simulink model "Unreal3DAnimation"  (R2026a)
settings: Solver=FixedStepAuto  StopTime=inf  FixedStep=0.02
undefined symbols (not defined in the file or in its folder): scenario, Sim3dSensor
libraries: sim3dlib x4, sim3dcameralib x2, dspvision x2, robotsim3dlib x1, visionsinks x1
settings Model: Creator=smaddina  LastModifiedBy=smaddina

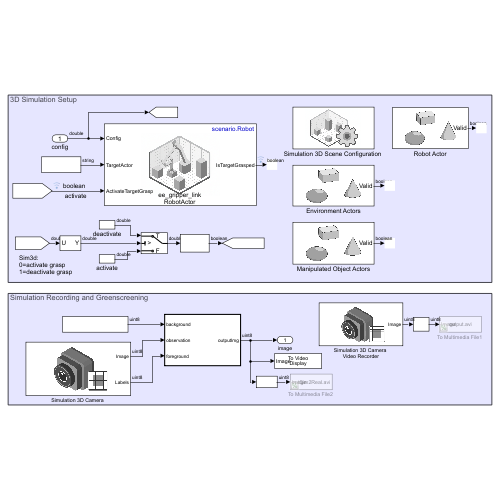
[thumbnail: Simulink's stored preview of the top-level diagram]
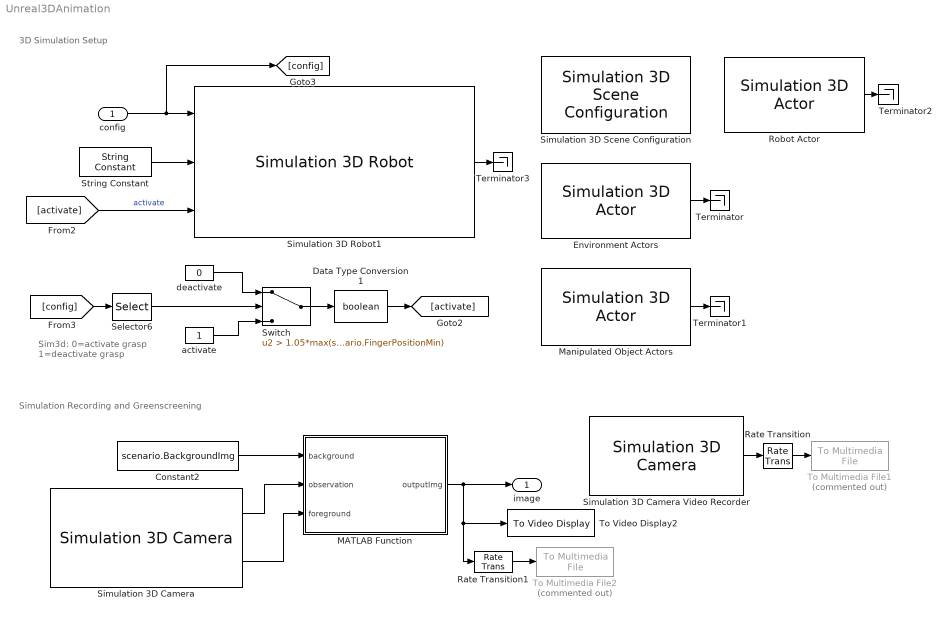
== system Unreal3DAnimation ==
  note: Simulation Recording and Greenscreening
  note: 3D Simulation Setup
  note: Sim3d:
      | 0=activate grasp
      | 1=deactivate grasp
  config : Inport  PortDimensions=scenario.NumConfig
  Constant2 : Constant  Value=scenario.BackgroundImg
  Data Type Conversion1 : DataTypeConversion  OutDataTypeStr=boolean  SaturateOnIntegerOverflow=off  RndMeth=Floor
  Environment Actors : sim3dlib/Simulation 3D Actor  Priority=1  ActorName=Sim3dActor1  ParentName=Scene Origin  Operation=Create at setup  InitScriptText=|  SampleTime=-1  Translation=[0 0 0]  Rotation=[0 0 0]  Scale=single([1 1 1])  aMode=5  ActorTag=Sim3dActor1  ActorType=Sim3dActor  ID=1
      | scenario = evalin("base", "scenario");
      | scenario.setupSceneActor(Actor, World)
  MATLAB Function : MATLAB Function  TreatAsAtomicUnit=on
  Manipulated Object Actors : sim3dlib/Simulation 3D Actor  Priority=1  ActorName=Sim3dActor2  ParentName=Scene Origin  Operation=Create at setup  InitScriptText=|  SampleTime=-1  Translation=[0 0 0]  Rotation=[0 0 0]  Scale=[1 1 1]  aMode=5  ActorTag=Sim3dActor2  ActorType=Sim3dActor  ID=2
      | scenario = evalin("base", "scenario");
      | scenario.setupObjectActor(Actor, World)
  Rate Transition : RateTransition  InitialCondition=zeros(scenario.ImageSize(1),scenario.ImageSize(2),3,'uint8')  OutPortSampleTime=0.2
  Rate Transition1 : RateTransition  InitialCondition=zeros(scenario.ImageSize(1),scenario.ImageSize(2),3,'uint8')  OutPortSampleTime=0.2
  Robot Actor : sim3dlib/Simulation 3D Actor  Priority=1  ActorName=Sim3dActor3  ParentName=Scene Origin  Operation=Create at setup  InitScriptText=|  SampleTime=-1  Translation=[0 0 0]  Rotation=[0 0 0]  Scale=[1 1 1]  aMode=5  ActorTag=Sim3dActor3  ActorType=Sim3dActor  ID=3
      | scenario = evalin("base", "scenario");
      | scenario.setupRobotActor(Actor, World)
  Selector6 : Selector  InputPortWidth=scenario.NumConfig  IndexOptions=Index vector (dialog)  Indices=scenario.FingerLinkIds(1)  OutputSizes=1
  "Simulation 3D Camera " : sim3dcameralib/Simulation 3D Camera  Priority=1  sensorTag=Sim3dSensor�  sensorId=1  sensorName=Sim3dSensor�  vehTagList={'RobotActor';'Scene Origin';'Sim3dActor1';'Sim3dActor2';'base_link'}  vehTag=RobotActor  CoordinateSystem=ISO8855  mountLoc=Origin  offsetFlag=on  tmountOffset=scenario.CameraTransl  extTmount=off  rmountOffset=scenario.CameraRot*180/pi  extRmount=off  FocalLength=scenario.FocalLength  OpticalCenter=scenario.OpticalCenter  ImageSize=scenario.ImageSize  RadialDistortion=[0, 0]  TangentialDistortion=[0, 0]  SensorSkew=0  VisualizeFieldOfView=off  FieldOfViewRange=61  DepthOutportEnabled=off  SemanticOutportEnabled=on  TransformOutportEnabled=off  SampleTime=-1  mountPoint=[0 -0.16 0.336]  mountOrientation=[2.40772307728316e-05 41.8103522312959 26.5650895133509]  aMode=6  ID=1
      settings: LibrarySourceBlock=robotsim3dlib/Simulation 3D Camera
  Simulation 3D Camera Video Recorder : sim3dcameralib/Simulation 3D Camera  Priority=1  sensorTag=Sim3dSensor�  sensorId=2  sensorName=Sim3dSensor�  vehTagList={'Custom ...';'RobotActor';'Scene Origin';'Sim3dActor1';'Sim3dActor2';'Sim3dActor3'}  vehTag=RobotActor  CoordinateSystem=ISO8855  mountLoc=Origin  offsetFlag=on  tmountOffset=scenario.CameraTransl*1.5+[-0.1,0,0]  extTmount=off  rmountOffset=scenario.CameraRot*180/pi  extRmount=off  FocalLength=scenario.FocalLength  OpticalCenter=scenario.OpticalCenter  ImageSize=scenario.ImageSize  RadialDistortion=[0, 0]  TangentialDistortion=[0, 0]  SensorSkew=0  VisualizeFieldOfView=off  FieldOfViewRange=61  DepthOutportEnabled=off  SemanticOutportEnabled=off  TransformOutportEnabled=off  SampleTime=-1  mountPoint=[-0.1 -0.24 0.504]  mountOrientation=[2.40772307728316e-05 41.8103522312959 26.5650895133509]  aMode=6  ID=2
      settings: LibrarySourceBlock=robotsim3dlib/Simulation 3D Camera
  Simulation 3D Robot1 : robotsim3dlib/Simulation 3D Robot  actorInputType=RigidBodyTree Object  RigidBodyTree=scenario.Robot  ActorName=RobotActor  existActorChekBox=on  initialTrans=[nan nan nan]  initialRot=[nan nan nan]  initialConfig=scenario.RobotInitConfig  EndEffector=ee_gripper_link  eeOffsetInpChekBox=off  eeTargetTrans=scenario.EndEffTargetTransl  eeTargetRot=[0 0 0]  enableRegionGraspChekBox=off  regionGraspInpChekBox=off  eeTargTransDiff=[0.2 0.2 0.2]  eeTargRotDiff=[0 0 0]  enableVisualVisualization=on  enableCollisionVisualization=off  collisionGeomColor=[0 1 0]  collisionGeomTransp=0.1  inpConfEnbVal=on  inpGraspEnbVal=on  inpTransEnbVal=off  outConfEnbVal=off  outGraspEnbVal=on  outTransEnbVal=off  SampleTime=-1  ActorType=SimulinkVehicle  ID=C  aMode=6  ActorTag=RobotActor  Mesh=RigidBodyTree
  "Simulation 3D Scene Configuration " : sim3dlib/Simulation 3D Scene Configuration  Priority=0  ProjectFormat=Default Scenes  SceneDesc=Empty scene  ProjectName=C:\Program Files\MATLAB\R2026a\toolbox\shared\sim3d_projects\automotive_project_windows\UE\WindowsNoEditor\VehicleSimulation.exe  ScenePath=/Game/Maps/EmptyScene  EnableOpenDRIVE=off  vehTagList={'Custom';'RobotActor';'Scene Origin';'Sim3dActor1';'Sim3dActor2';'Sim3dActor3'}  vehTag=Custom  AttachedCameraRelativeTranslation=[0 0 0]  FreeCameraDefaultInitialTranslation=[-6, 0, 2]  AttachedCameraRelativeRotation=[0, -15, 0]  FreeCameraDefaultInitialRotation=[0, -15, 0]  ViewpointName=Custom  FreeCameraInitialTranslation=[0.8 -0.2 1.5]  FreeCameraInitialRotation=[0 -28.64789 -180]  OpVisEn=off  Ts=0.02  EnableWindow=on  EnableRemoteAccess=off  SimulationMode=CoSimulation  SimulateUsing=Interpreted execution  EnableAnimationRecording=off  OverrideDefaultRecording=off  AnimationRecordingFileName=sim3dAnimation.mat  AnimationRecordingInterval=[0 inf]  EnableWeather=on  SunAzimuth=40  SunAltitude=19.800  EnableGeospatialSun=off  Latitude=0  Longitude=0  Date=2023-01-01  Time=10:30:00  GeoTimeZone=-5.0  SunDaylightSaving=off  wind=1  clouds=10  EnableVolumetricClouds=off  CloudCoverage=0  CloudAltitude=6  fog=0  rain=0  RaindropsEffect=off  SnowDensity=0  EnableGeospatial=off  TilesetSource=Earth terrain  UseTrueOrigin=off  OriginHeight=200  OriginLatitude=40.744652  OriginLongitude=-73.988864  MapStyle=Aerial  AdditionalAssetIDs=[]  UseAdvancedSunSky=off  SolarTime=11  TimeZone=-5  Day=21  Month=9  Year=2022  UseDaylightSavingTime=on  DSTStartDay=10  DSTStartMonth=3  DSTEndDay=3  DSTEndMonth=11  DSTSwitchHour=2  sensorTag=MainCamera1  sensorId=1  sensorName=MainCamera1  mountLoc=Origin  offsetFlag=off  tmountOffset=[0, 0, 0]  rmountOffset=[0, 0, 0]  HorizontalResolution=1280  VerticalResolution=720  HorizontalFOV=60  mountPoint=[0 0 0]  mountOrientation=[0 0 0]  aMode=6  ID=1  GeoTrigger=Inactive  ViewNameList={'Custom'}  ViewTranslationList={'[0.8 -0.2 1.5]'}  ViewRotationList={'[0 -28.64789 -180]'}
      settings: LibrarySourceBlock=robotsim3dlib/Simulation 3D Scene Configuration
  String Constant : StringConstant  String="\"targetActor\""
  Switch : Switch  Criteria=u2 > Threshold  Threshold=1.05*max(scenario.FingerClose, scenario.FingerPositionMin)  SaturateOnIntegerOverflow=off  InputSameDT=off
  Terminator{,1..3} (4 alike) : Terminator
  "To Multimedia File1 " : dspvision/To Multimedia File  Commented=on  outputFilename=output.avi  streamSelection=Video only  videoCompressor=None (uncompressed)  audioCompressor=None (uncompressed)  imagePorts=One multidimensional signal  fileType=AVI  audioDatatype=Determine from input data type  fourcc=RGB  audioBitRate=128  audioQuality=75  videoQuality=75  mj2000CompFactor=10
      settings: LibrarySourceBlock=visionsinks/To Multimedia File
  "To Multimedia File2 " : dspvision/To Multimedia File  Commented=on  outputFilename=outSim2Real.avi  streamSelection=Video only  videoCompressor=None (uncompressed)  audioCompressor=None (uncompressed)  imagePorts=One multidimensional signal  fileType=AVI  audioDatatype=Determine from input data type  fourcc=RGB  audioBitRate=128  audioQuality=75  videoQuality=75  mj2000CompFactor=10
      settings: LibrarySourceBlock=visionsinks/To Multimedia File
  To Video Display2 : visionsinks/To Video Display  windowSizeMode=Normal  openAtMdlStart=on  fullScreen=off  videoWindowX=793  videoWindowY=307  saveWindowSize=off  videoWindowWidth=870  videoWindowHeight=553  inputColorFormat=RGB  inputType=Obsolete  imagePorts=One multidimensional signal  OutputDevice=On-screen video monitor  dataOrg=Column-major  isWindowOpen=off
  activate : Constant
  deactivate : Constant  Value=0
  image : Outport  PortDimensions=[scenario.ImageSize,3]
  wires:
  Environment Actors/1 -> Terminator/1
  config/1 -> [config], Simulation 3D Robot1/1
  "Simulation 3D Camera "/2 -> MATLAB Function/3(foreground)
  [config] -> Selector6/1
  Switch/1 -> Data Type Conversion1/1
  Data Type Conversion1/1 -> [activate]
  activate/1 -> Switch/3
  deactivate/1 -> Switch/1
  Manipulated Object Actors/1 -> Terminator1/1
  Robot Actor/1 -> Terminator2/1
  Constant2/1 -> MATLAB Function/1(background)
  "Simulation 3D Camera "/1 -> MATLAB Function/2(observation)
  Selector6/1 -> Switch/2
  String Constant/1 -> Simulation 3D Robot1/2
  [activate] -> Simulation 3D Robot1/3  "activate"
  MATLAB Function/1(outputImg) -> Rate Transition1/1, To Video Display2/1, image/1
  Rate Transition/1 -> "To Multimedia File1 "/1
  Rate Transition1/1 -> "To Multimedia File2 "/1
  Simulation 3D Robot1/1 -> Terminator3/1
  Simulation 3D Camera Video Recorder/1 -> Rate Transition/1

== matlab function Unreal3DAnimation/MATLAB Function ==
  data: background input; observation input; outputImg output; foreground input
function outputImg = sim2real(background, observation, foreground)


foregroundMask = uint8(foreground~=0);
outputImg = observation.*foregroundMask + background.*(1-foregroundMask);
